simulink model "pvwindupfc11"  (R2016a)
settings: Solver=VariableStepAuto  StartTime=0.0  StopTime=0.5  RelTol=1e-3
undefined symbols (not defined in the file): BCMS11, c1, c2, c3, c4, c5, c6, Clink_3L, DiscIntNeverNeededParam, fdesignblkfcn, Fnom, gcbh, Ion, Ki_Ireg_3L, Ki_VDCreg_3L, Kp_Ireg_3L, Kp_VDCreg_3L, LimitL_Ireg_3L, LimitL_VDCreg_3L, LimitU_Ireg_3L, LimitU_VDCreg_3L, Lithium, LowerLimit, Pnom_3L, Pnom_dc_3L, PV11, Ts_Control, Ts_Power, Ts_PWM, UpperLimit, Vnom_dc_3L, Vnom_prim_3L, Vnom_sec_3L
libraries: powerlib x98, powerlib_extras x29, powerlib_meascontrol x20, fuzblock x2, simulink x1, electricdrivelib x1
(part 2 of 4)

== system pvwindupfc11/100Vdc DC//DC Converter1 ==
  Add : Sum
  CBus : powerlib/Elements/Series RLC Branch  LConnTagsString=__new0  RConnTagsString=__new0  BranchType=RC  Resistance=0.2  Inductance=1e-3  SetiL0=off  InitialCurrent=0  Capacitance=7500e-6  Setx0=on  InitialVoltage=100  Measurements=None
  Chopper : Subsystem  mask(SPSdrives Converter){SnubberResistance=10e3, SnubberCapacitance=inf, Ron=1e-3, ForwardVoltages=[1.3,1.3], IGBTParameters=[0,0], converterType=Inverter}
      mask prompts: SnubberResistance "Snubber resistance Rs (Ohms):"; SnubberCapacitance "Snubber capacitance Cs (F):"; Ron "Ron (Ohms):"; ForwardVoltages "Forward voltages [Device Vf(V), Diode Vd (V)]"; IGBTParameters "[Tf(s), Tt(s)]:"; converterType "Converter type:"
      mask help: This model implements an average-value buck converter."Duty Cycle" contains the duty cycle of the internal IGBT device.
      mask TypeOptions converterType: Rectifier | Inverter
      mask Display: plot(0,0,100,100,[39 39 23.8],[71 28 28],[44 56 49.6 56 52.8 56 61 61],[39.2 33.6 32.8 33.6 40.8 33.6 30 12.4],[44 44 44 61 61],[28 71 60 66.4 90],[75 67 83 75 67 83 75 75],[54 42 42 54 54 54 54 66],[61 75 75],[24 24 42],[75 75 61],[66,76,76])
  Constant : Constant  Value=100
  Current controller DISCRETE1 : Subsystem  mask(PI controller){Kp=0.0005, Ki=0.15, Ts=1e-3}
      mask prompts: Kp "Proportional gain (Kp)"; Ki "Integral gain (Ki)"; Ts "Sample time (s) :"
      mask help: Proportional-Integral Speed Controller
      mask Display: plot(0,0,100,100,[35,35,65],[70,30,30],[35,65],[45,60])
  Current controller DISCRETE2 : Subsystem  mask(PI controller){Kp=0.0005, Ki=0.15, Ts=1e-3}
      mask prompts: Kp "Proportional gain (Kp)"; Ki "Integral gain (Ki)"; Ts "Sample time (s) :"
      mask help: Proportional-Integral Speed Controller
      mask Display: plot(0,0,100,100,[35,35,65],[70,30,30],[35,65],[45,60])
  Duty Cycles : Subsystem
  L : powerlib/Elements/Series RLC Branch  LConnTagsString=__new0  RConnTagsString=__new0  BranchType=L  Resistance=0.3  Inductance=500e-6  SetiL0=off  InitialCurrent=0  Capacitance=100e-6  Setx0=off  InitialVoltage=0  Measurements=None
  Timer : Subsystem  DialogController=POWERSYS.PowerSysDialog  mask(Timer){t=[ 0  1], e=[1 1 ]}
      mask prompts: t "Time (s):"; e "Amplitude:"
      mask help:
      | Generates a signal changing at specified times.
      |
      | If a signal value is not specified at time zero, the output is kept at 0 until the first specified transition time.
      mask init:
      | tt=t;
      | sv=e;
      | if isempty(tt) | isempty(sv)
      | 	% probably during the load process when under a masked block.
      | 	tt=0;
      | 	sv=1;
      | end
      | %
      | if length(sv) ~= length(tt),
      |    Erreur.message = 'The vectors specifying the time and amplitude pairs must have the same length.';
      |    Erreur.identifier = 'SimPowerSystems:TimerBlock:ParameterError';
      |    powericon('psberror',Erreur.message,Erreur.identifier,'NoUiwait');
      | end
      | if tt(1)~=0,
      |    tt=[0 tt];
      |    sv=[~sv(1) sv];
      | end
      | n=length(tt);
      | vec_dt=[tt,0]-[0,tt] ;
      | vec_dt=vec_dt(2:n);
      | if any(vec_dt<=0)
      |    Erreur.message = 'All transition times must be in increasing order.';
      |    Erreur.identifier = 'SimPowerSystems:TimerBlock:ParameterError';
      |    powericon('psberror',Erreur.message,Erreur.identifier,'NoUiwait');
      | end
      | tv=[-1,tt(1),reshape(repmat(reshape(tt(2:end),1,length(tt)-1),2,1),1,2*length(tt)-2),tt(end)+1];
      | %sv=(sv(:)'~=0);
      | opv=[sv(1),reshape(repmat(sv(1:end-1),2,1),1,2*length(sv)-2),sv(end),sv(end)];
      | 
      | power_initmask();
      mask Help: web(psbhelp)
      mask Display: plot( tv(2:end-1), opv(2:end-1) )
  Transfer Fcn : TransferFcn  Denominator=[0.001 1]
  Voltage Measurement : powerlib/Measurements/Voltage Measurement  PhasorSimulation=off  OutputType=Complex  PSBequivalent=0
  + : PMIOPort  Tag=PMCPort  Port=1  Side=Right
  - : PMIOPort  Tag=PMCPort  Port=2  Side=Right
  + input : PMIOPort  Tag=PMCPort  Port=3  Side=Left
  -input : PMIOPort  Tag=PMCPort  Port=4  Side=Left
  wires:
  Transfer Fcn/1 -> Current controller DISCRETE1/1(UBus)
  Duty Cycles/1(dc) -> Chopper/1(Duty Cycle)
  Voltage Measurement/1 -> Transfer Fcn/1
  Constant/1 -> Current controller DISCRETE1/2(Uref)
  Timer/1(Out) -> Current controller DISCRETE2/1(Pref)
  [Ppv] -> Current controller DISCRETE2/2(Ppv)
  Current controller DISCRETE2/1(Delta Ec) -> Add/2
  Add/1 -> Duty Cycles/1(Ec)
  Current controller DISCRETE1/1(Ec) -> Add/1
  connections:
  + input/RConn1 -- L/RConn1
  Chopper/RConn1 -- L/LConn1
  CBus/LConn1 -- Chopper/LConn1 -- +/RConn1 -- Voltage Measurement/LConn1
  Chopper/LConn2 -- CBus/RConn1 -- -/RConn1 -- Voltage Measurement/LConn2 -- -input/RConn1

== system pvwindupfc11/60 kW  PV Array 1 ==
  note: Diode characteristic
      |    Id=Isat*[exp(Vd/VT) -1]
      |
      | where:
      |    Id = diode cuurent (A)
      |    Vd = diode voltage (V)
      |  Isat = diode saturation current (A)
      |    VT = temperature voltage = k*T/q*Qd*Ncell*Nser
      |
      |     T = cell temperature (K),
      |     k = Boltzman constant = 1.3806e-23 J.K^-1
      |     q = electron charge = 1.6022e-19 C
      |    Qd = diode quality factor
      |  Ncell= number of series-connected cells per module
      |  Nser = number of series-connected modules per string
  Ir : Inport
  Add : Sum  Inputs=+-
  Bus Creator : BusCreator  Inputs=4
  Diode : Subsystem
      mask Display:
      | plot(-75,-50,100,150, [-15 -15 43 -15 -15 -75],[50 8 50 92 50 50], ...
      |     [43 43],[8 94],[100 43], [50 50])
  I_PV : powerlib/Measurements/Current Measurement  PhasorSimulation=off  OutputType=Complex  PSBequivalent=0
  Iph : powerlib/Electrical Sources/Controlled Current Source  Initialize=on  Source_Type=AC  Amplitude=0  Phase=0  Frequency=0  Measurements=None
  Iph_ : Constant  Value=Iph_array
  Product1 : Product  Inputs=**  RndMeth=Zero
  Rp : powerlib/Elements/Series RLC Branch  LConnTagsString=__new0  RConnTagsString=__new0  BranchType=R  Resistance=Rp_array  Inductance=1e-3  SetiL0=off  InitialCurrent=0  Capacitance=1e-6  Setx0=off  InitialVoltage=0  Measurements=Branch current
  Rs : powerlib/Elements/Series RLC Branch  LConnTagsString=__new0  RConnTagsString=__new0  BranchType=R  Resistance=Rs_array  Inductance=1e-3  SetiL0=off  InitialCurrent=0  Capacitance=1e-6  Setx0=off  InitialVoltage=0  Measurements=None
  Rs_ : Gain  Gain=Rs_array
  t0_kW : Gain  Gain=1e-3
  + : PMIOPort  Port=1  Side=Right
  - : PMIOPort  Port=2  Side=Right
  m : Outport
  wires:
  Product1/1 -> Iph/1
  Iph_/1 -> Product1/1
  Ir/1 -> t0_kW/1, Bus Creator/4  "Irradiance (W/m^2)"
  Diode/1(Vdiode) -> Add/1  "Vdiode"
  Rs_/1 -> Add/2
  I_PV/1 -> Rs_/1, Bus Creator/2  "I_PV"
  t0_kW/1 -> Product1/2
  Add/1 -> Bus Creator/1  "V_PV"
  Diode/2(Idiode) -> Bus Creator/3  "I_diode"
  Bus Creator/1 -> m/1
  connections:
  Iph/LConn1 -- Diode/RConn1 -- -/RConn1 -- Rp/RConn1
  Diode/LConn1 -- Iph/RConn1 -- Rs/RConn1 -- Rp/LConn1
  Rs/LConn1 -- I_PV/LConn1
  +/RConn1 -- I_PV/RConn1

== system pvwindupfc11/Control Systems  ==
  REC Control : Subsystem
  SEC Control : Subsystem

== system pvwindupfc11/Control of Inverter ==
  note: Control of Inverter
  Discrete PWM Generator1 : Subsystem  AncestorBlock=|  DialogController=POWERSYS.PowerSysDialog  mask(Discrete PWM Generator){GeneratorMode=3-arm  bridge (6 pulses), Fc=4000, Ts=50e-6, Internal=off, mIndex=0.99, Freq=50, Phase=0}
      | powerlib_extras/Discrete 
      | Control Blocks/Discrete
      | PWM Generator
      mask prompts: GeneratorMode "Generator Mode"; Fc "Carrier frequency (Hz):"; Ts "Sample time:"; Internal "Internal generation of modulating signal(s)"; mIndex "Modulation index  (0<m<1) :"; Freq "Frequency of output voltage (Hz)"; Phase "Phase of output voltage (degrees)"
      mask help:
      | This discrete block generates pulses for carrier-based PWM (Pulse Width Modulation), self-commutated IGBTs,GTOs or FETs bridges.
      |
      | Depending on the number of bridge arms selected in the "Generator Mode" parameter, the block can be used either for single-phase or three-phase PWM control.
      mask init:
      | powericon('psbcallbacks',gcb,'Discrete PWM Generator');
      | if Freq==0
      |     Phase=90;
      | end
      | switch GeneratorMode
      | case 1,
      |     Internal_Phase=0;
      |    Signal_PortWidth=1;
      |    Select1_Elements=[1 2];
      |    Select1_PortWidth=2;
      |    Select3_Elements=[1 2];
      |    Select3_PortWidth=4;
      | case 2,
      |     Internal_Phase=0;
      |     Signal_PortWidth=1;
      |     Select1_Elements=[1 2];
      |     Select1_PortWidth=2;
      |     Select3_Elements=[1 2 3 4];
      |     Select3_PortWidth=4;
      | case 3,
      |     Internal_Phase=[0 -2*pi/3 2*pi/3];
      |     Signal_PortWidth=3;
      |     Select1_Elements=[1 4 2 5 3 6];
      |     Select1_PortWidth=6;
      |    Select3_Elements=[1 2 3 4 5 6];
      |    Select3_PortWidth=12;
      | case 4,
      |     Internal_Phase=[0 -2*pi/3 2*pi/3];
      |     Signal_PortWidth=3;
      |     Select1_Elements=[1 4 2 5 3 6];
      |     Select1_PortWidth=6;
      |    Select3_Elements=[1 2 3 4 5 6 7 8 9 10 11 12];
      |    Select3_PortWidth=12;
      | end
      | power_initmask();
      mask Help:
      | The output pulses are a vector (with values=0 or 1). Depending on the selected "Generator Mode", the output vector contains:
      | For a 1-arm  bridge: Two pulses. Pulse 1 is for the upper switch and pulse 2 is for the lower switch.
      | For a 2-arm  bridge: Four pulses. Pulses 1 and 3 are respectively for the upper switches of the first and second arm. Pulses 2 and 4 are for the lower switches.
      | For a 3-arm  bridge: Six pulses. Pulses 1,3 and 5 are respectively for the upper switches of the first,second and third arm. Pulses 2,4 and 6 are for the lower switches.
      | For double 3-arm bridges: Twelve pulses.The first six pulses (pulses 1 to 6) must be sent to the first 3-arm bridge and the last six (pulses 7 to 12) to the second 3-arm bridge.
      | 
      | By selecting "Internal generation" you can can control the modulation index m, frequency and phase of the output voltage  from the internal parameters (m, Freq and Phase). Otherwise, external signals are used for pulse generation. The width of the input vector must be 1 for single phase bridges ( 1-arm or 2-arm)  and 3 for 3-phase bridges  (single or double bridge).
      mask TypeOptions GeneratorMode: 1-arm  bridge (2 pulses) | 2-arm  bridge (4 pulses) | 3-arm  bridge (6 pulses) | Double 3-arm  bridges (12 pulses)
      mask Callback Internal: powericon('psbcallbacks',gcb,'Discrete PWM Generator',[]);
  MI Controller : Subsystem
  Subsystem1 : Subsystem
  Unit Delay4 : UnitDelay  SampleTime=20e-6
  VL-L : Scope
  Vph_rms : Scope
  m : Scope
  C : PMIOPort  Port=1  Side=Left
  B : PMIOPort  Port=2  Side=Left
  A : PMIOPort  Port=3  Side=Left
  Pulses : Outport
  wires:
  MI Controller/2(m) -> m/1
  Unit Delay4/1 -> Pulses/1
  Subsystem1/1(Vph) -> MI Controller/1(Vabc)
  Subsystem1/2(VL-L) -> VL-L/1
  Subsystem1/3(Vph_rms) -> Vph_rms/1
  Discrete PWM Generator1/1(Pulses) -> Unit Delay4/1
  MI Controller/1(Vabc_inv) -> Discrete PWM Generator1/1(Uref)
  connections:
  A/RConn1 -- Subsystem1/LConn1
  B/RConn1 -- Subsystem1/LConn2
  C/RConn1 -- Subsystem1/LConn3

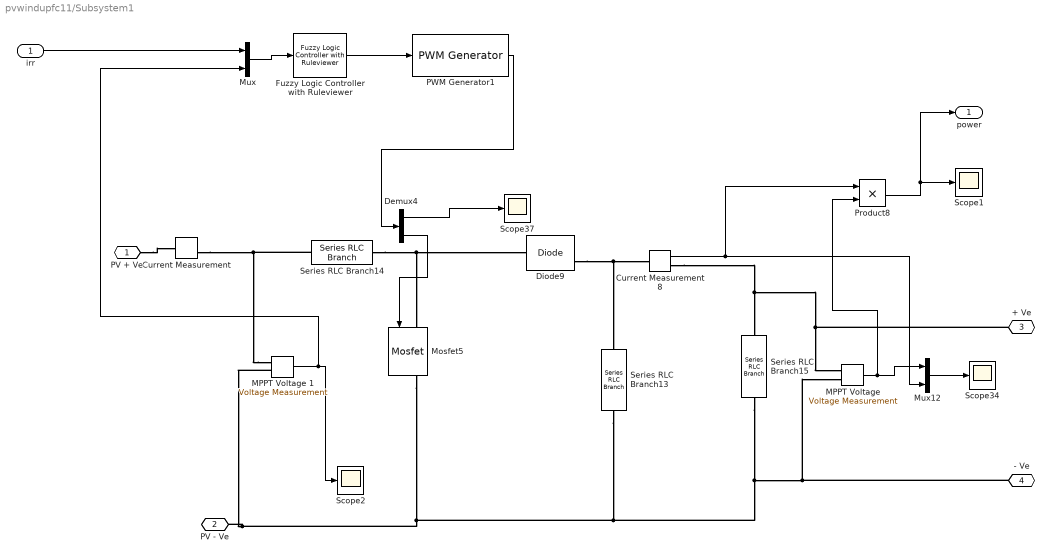
== system pvwindupfc11/Subsystem1 ==
  irr : Inport
  Current Measurement : powerlib/Measurements/Current Measurement  PhasorSimulation=off  OutputType=Complex  PSBequivalent=0
  Current Measurement8 : powerlib/Measurements/Current Measurement  PhasorSimulation=off  OutputType=Complex  PSBequivalent=0
  Demux4 : Demux  Outputs=2
  Diode9 : powerlib/Power Electronics/Diode  Ron=0.001  Lon=0  Vf=0.8  IC=0  UseSnubber=off  Rs=500  Cs=250e-9  Measurements=on
  Fuzzy Logic Controller with Ruleviewer : fuzblock/Fuzzy Logic  Controller  with Ruleviewer  fismatrix=[PV11]  Ts=0.01
  "MPPT Voltage " : powerlib/Measurements/Voltage Measurement  PhasorSimulation=off  OutputType=Complex  PSBequivalent=0
  MPPT Voltage 1 : powerlib/Measurements/Voltage Measurement  PhasorSimulation=off  OutputType=Complex  PSBequivalent=0
  Mosfet5 : powerlib/Power Electronics/Mosfet  Ron=0.1  Lon=0  Rd=0.01  Vfd=0  IC=0  Rs=1e5  Cs=inf  Measurements=on
  Mux : Mux  Inputs=2
  Mux12 : Mux  Inputs=2
  PWM Generator1 : powerlib_extras/Control  Blocks/PWM Generator  GeneratorMode="1-arm  bridge (2 pulses)"  Fc=2000  Internal=off  mIndex=0.4  Freq=50  Phase=0
  Product8 : Product  RndMeth=Zero
  Scope{1..2,34,37} (4 alike) : Scope
  Series RLC Branch13 : powerlib/Elements/Series RLC Branch  LConnTagsString=__new0  RConnTagsString=__new0  BranchType=C  Resistance=1  Inductance=1e-3  SetiL0=off  InitialCurrent=0  Capacitance=15.5e-4  Setx0=off  InitialVoltage=0  Measurements=None
  Series RLC Branch14 : powerlib/Elements/Series RLC Branch  LConnTagsString=__new0  RConnTagsString=__new0  BranchType=L  Resistance=1  Inductance=0.05e-2  SetiL0=off  InitialCurrent=0  Capacitance=1e-6  Setx0=off  InitialVoltage=0  Measurements=None
  Series RLC Branch15 : powerlib/Elements/Series RLC Branch  LConnTagsString=__new0  RConnTagsString=__new0  BranchType=R  Resistance=55  Inductance=1e-3  SetiL0=off  InitialCurrent=0  Capacitance=1e-6  Setx0=off  InitialVoltage=0  Measurements=None
  PV + Ve : PMIOPort  Port=1  Side=Left
  PV - Ve : PMIOPort  Port=2  Side=Left
  + Ve : PMIOPort  Port=3  Side=Right
  - Ve : PMIOPort  Port=4  Side=Right
  "power " : Outport
  wires:
  Demux4/2 -> Mosfet5/1
  PWM Generator1/1 -> Demux4/1
  Demux4/1 -> Scope37/1
  Mux12/1 -> Scope34/1
  "MPPT Voltage "/1 -> Product8/2, Mux12/1
  Current Measurement8/1 -> Product8/1, Mux12/2
  Product8/1 -> "power "/1, Scope1/1
  MPPT Voltage 1/1 -> Mux/2, Scope2/1
  Fuzzy Logic Controller with Ruleviewer/1 -> PWM Generator1/1
  Mux/1 -> Fuzzy Logic Controller with Ruleviewer/1
  irr/1 -> Mux/1
  connections:
  MPPT Voltage 1/LConn1 -- Series RLC Branch14/LConn1 -- Current Measurement/RConn1
  MPPT Voltage 1/LConn2 -- PV - Ve/RConn1 -- Series RLC Branch13/RConn1 -- - Ve/RConn1 -- "MPPT Voltage "/LConn2 -- Series RLC Branch15/RConn1 -- Mosfet5/RConn1
  + Ve/RConn1 -- Series RLC Branch15/LConn1 -- Current Measurement8/RConn1 -- "MPPT Voltage "/LConn1
  Diode9/RConn1 -- Current Measurement8/LConn1 -- Series RLC Branch13/LConn1
  Series RLC Branch14/RConn1 -- Diode9/LConn1 -- Mosfet5/LConn1
  PV + Ve/RConn1 -- Current Measurement/LConn1

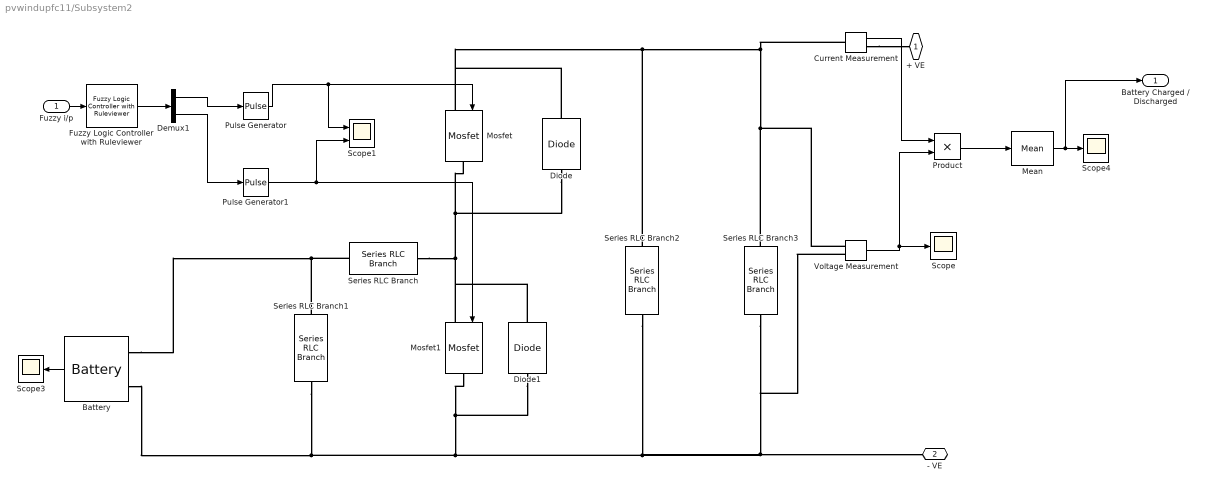
== system pvwindupfc11/Subsystem2 ==
  Fuzzy i/p : Inport
  Battery : electricdrivelib/Extra Sources/Battery  BatType=Lithium-Ion  ShowTempParam=off  ThermalPreset=no  NomV=440  NomQ=30  SOC=100  Batt_Tr=1  PresetModel=off  MaxQ=30  MinV=330  FullV=512.1543  Dis_rate=13.0435  R=0.14667  Normal_OP=27.1304  expZone="[475.3698      1.473913]"  current=[6.5 13 32.5]  Units=Time  Tci=20  NomT=25  T2=0  MaxQ2=2.208  FullV2=3.45  Normal_OP2=2.8  expZone2="[3.22        0.23]"  Rca=0.6  ti=1000  Dp=0
  Current Measurement : powerlib/Measurements/Current Measurement  PhasorSimulation=off  OutputType=Complex  PSBequivalent=0
  Demux1 : Demux  Outputs=2
  Diode : powerlib/Power Electronics/Diode  Ron=0.001  Lon=0  Vf=0.8  IC=0  UseSnubber=off  Rs=500  Cs=250e-9  Measurements=off
  Diode1 : powerlib/Power Electronics/Diode  Ron=0.001  Lon=0  Vf=0.8  IC=0  UseSnubber=off  Rs=500  Cs=250e-9  Measurements=off
  Fuzzy Logic Controller with Ruleviewer : fuzblock/Fuzzy Logic  Controller  with Ruleviewer  fismatrix=[BCMS11]  Ts=0.1
  Mean : powerlib_meascontrol/Measurements/Mean  Freq=60  Vinit=0  Ts=0
  Mosfet : powerlib/Power Electronics/Mosfet  Ron=0.1  Lon=0  Rd=0.01  Vfd=0  IC=0  Rs=1e5  Cs=inf  Measurements=off
  Mosfet1 : powerlib/Power Electronics/Mosfet  Ron=0.1  Lon=0  Rd=0.01  Vfd=0  IC=0  Rs=1e5  Cs=inf  Measurements=off
  Product : Product
  Pulse Generator : DiscretePulseGenerator  PulseType=Time based  TimeSource=Use external signal  Period=0.01  PulseWidth=99  PhaseDelay=0.001
  Pulse Generator1 : DiscretePulseGenerator  PulseType=Time based  TimeSource=Use external signal  Period=0.01  PulseWidth=99  PhaseDelay=0.001
  Scope : Scope
  Scope1 : Scope  NumInputPorts=2
  Scope3 : Scope
  Scope4 : Scope
  Series RLC Branch : powerlib/Elements/Series RLC Branch  LConnTagsString=__new0  RConnTagsString=__new0  BranchType=L  Resistance=1  Inductance=100e-6  SetiL0=off  InitialCurrent=0  Capacitance=1e-6  Setx0=off  InitialVoltage=0  Measurements=None
  Series RLC Branch1 : powerlib/Elements/Series RLC Branch  LConnTagsString=__new0  RConnTagsString=__new0  BranchType=RC  Resistance=1  Inductance=1e-3  SetiL0=off  InitialCurrent=0  Capacitance=700e-4  Setx0=off  InitialVoltage=0  Measurements=None
  Series RLC Branch2 : powerlib/Elements/Series RLC Branch  LConnTagsString=__new0  RConnTagsString=__new0  BranchType=RC  Resistance=2  Inductance=1e-3  SetiL0=off  InitialCurrent=0  Capacitance=700e-4  Setx0=off  InitialVoltage=0  Measurements=None
  Series RLC Branch3 : powerlib/Elements/Series RLC Branch  LConnTagsString=__new0  RConnTagsString=__new0  BranchType=R  Resistance=0.3  Inductance=1e-3  SetiL0=off  InitialCurrent=0  Capacitance=1e-6  Setx0=off  InitialVoltage=0  Measurements=None
  Voltage Measurement : powerlib/Measurements/Voltage Measurement  PhasorSimulation=off  OutputType=Complex  PSBequivalent=0
  + VE : PMIOPort  Port=1  Side=Right
  - VE : PMIOPort  Port=2  Side=Right
  "Battery Charged / Discharged " : Outport
  wires:
  Battery/1 -> Scope3/1
  Fuzzy Logic Controller with Ruleviewer/1 -> Demux1/1
  Demux1/1 -> Pulse Generator/1
  Demux1/2 -> Pulse Generator1/1
  Voltage Measurement/1 -> Product/2, Scope/1
  Pulse Generator1/1 -> Scope1/2, Mosfet1/1
  Pulse Generator/1 -> Scope1/1, Mosfet/1
  Fuzzy i/p/1 -> Fuzzy Logic Controller with Ruleviewer/1
  Current Measurement/1 -> Product/1
  Product/1 -> Mean/1
  Mean/1 -> "Battery Charged / Discharged "/1, Scope4/1
  connections:
  Series RLC Branch/RConn1 -- Mosfet1/LConn1 -- Diode1/RConn1 -- Diode/LConn1 -- Mosfet/RConn1
  Series RLC Branch/LConn1 -- Series RLC Branch1/LConn1 -- Battery/LConn1
  Mosfet1/RConn1 -- Diode1/LConn1 -- Battery/LConn2 -- Series RLC Branch1/RConn1 -- Series RLC Branch2/RConn1 -- Series RLC Branch3/RConn1 -- Voltage Measurement/LConn2 -- - VE/RConn1
  Series RLC Branch3/LConn1 -- Current Measurement/LConn1 -- Diode/RConn1 -- Mosfet/LConn1 -- Series RLC Branch2/LConn1 -- Voltage Measurement/LConn1
  Current Measurement/RConn1 -- + VE/RConn1

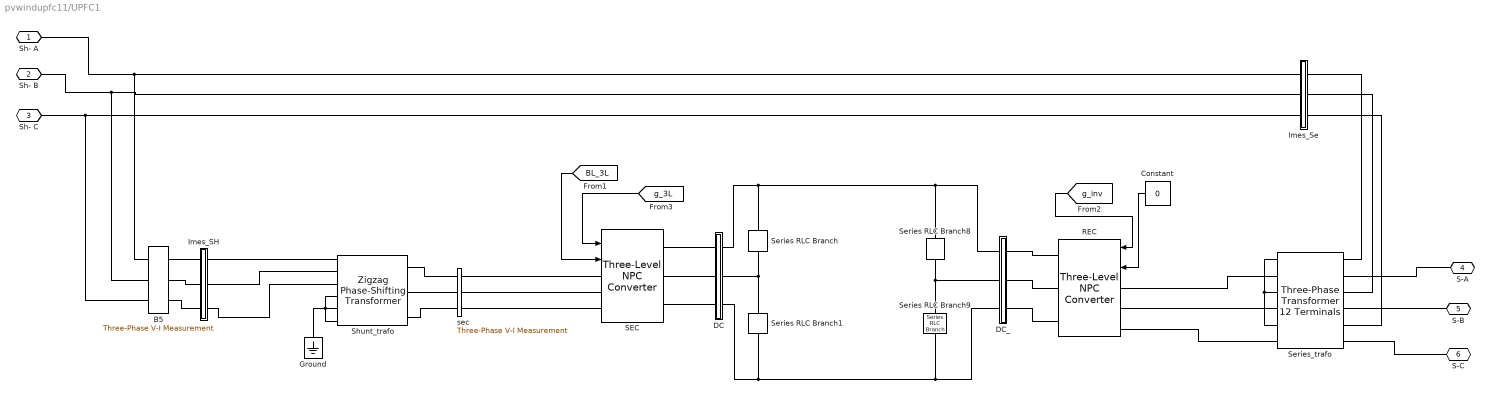
== system pvwindupfc11/UPFC1 ==
  B5 : powerlib/Measurements/Three-Phase V-I Measurement  VoltageMeasurement=phase-to-phase  SetLabelV=on  LabelV=V_shunt  Vpu=off  VpuLL=off  CurrentMeasurement=yes  SetLabelI=on  LabelI=i_shunt_  Ipu=off  Pbase=100e6  Vbase=500e3  OutputType=Complex  PhasorSimulation=off  PSBequivalent=0
  Constant : Constant  Value=0
  DC : Subsystem
  DC_ : Subsystem
  Ground : powerlib/Elements/Ground  LConnTagsString=a
  Imes_SH : Subsystem
  Imes_Se : Subsystem
  REC : powerlib/Power Electronics/Three-Level NPC Converter  ModelType=Switching devices  Ron=1e-3  Rs=1e6  Cs=inf  Vforward=[0,0]  Ron_Diode=1e-3  Rs_Diode=1e6  Cs_Diode=inf  Vf_Diode=1e-3  Rs_CurrentSource=inf
  SEC : powerlib/Power Electronics/Three-Level NPC Converter  ModelType=Switching devices  Ron=1e-3  Rs=1e6  Cs=inf  Vforward=[ 0, 0 ]  Ron_Diode=1e-3  Rs_Diode=1e6  Cs_Diode=inf  Vf_Diode=1e-3  Rs_CurrentSource=inf
      settings: AttributesFormatString=%<ModelType>
  Series RLC Branch : powerlib/Elements/Series RLC Branch  LConnTagsString=__new0  RConnTagsString=__new0  BranchType=C  Resistance=1  Inductance=1e-3  SetiL0=off  InitialCurrent=0  Capacitance=Clink_3L  Setx0=on  InitialVoltage=Vc_Initial_3L  Measurements=None
  Series RLC Branch1 : powerlib/Elements/Series RLC Branch  LConnTagsString=__new0  RConnTagsString=__new0  BranchType=C  Resistance=1  Inductance=1e-3  SetiL0=off  InitialCurrent=0  Capacitance=Clink_3L  Setx0=on  InitialVoltage=Vc_Initial_3L  Measurements=None
  Series RLC Branch8 : powerlib/Elements/Series RLC Branch  LConnTagsString=__new0  RConnTagsString=__new0  BranchType=C  Resistance=1  Inductance=1e-3  SetiL0=off  InitialCurrent=0  Capacitance=Clink_3L  Setx0=on  InitialVoltage=Vc_Initial_3L  Measurements=None
  Series RLC Branch9 : powerlib/Elements/Series RLC Branch  LConnTagsString=__new0  RConnTagsString=__new0  BranchType=C  Resistance=1  Inductance=1e-3  SetiL0=off  InitialCurrent=0  Capacitance=Clink_3L  Setx0=off  InitialVoltage=1000  Measurements=None
  Series_trafo : powerlib/Elements/Three-Phase Transformer 12 Terminals  RatedPower="[Pnom_3L,  Fnom ]"  Winding1="[Vnom_sec_3L   0.002  0.1/2]"  Winding2="[Vnom_sec_3L   0.002  0.1/2]"  RmXm=[ 500 500 ]
  Shunt_trafo : powerlib/Elements/Zigzag Phase-Shifting Transformer  SecondaryConnection=Y  UNITS=SI  NominalPower="[Pnom_3L,  Fnom ]"  PrimaryVoltage=Vnom_prim_3L  SecondaryVoltage="[Vnom_sec_3L   1]"  Winding1=[1.0624 0.084547]  Winding2=[0.00042304 3.3664e-05]  Winding3=[0.0004 3.1831e-05]  SetSaturation=off  RmLm=[3.1873e+05 3.1873e+05]  Rm=3.1873e+05  Saturation=[0 0;0.077613 65.62;32.339 83.118]  SetInitialFlux=off  Measurements=None  InitialFluxes=[0 0 0]  MoreParameters=off  BreakLoop=off  DataType=on
      settings: AttributesFormatString=\n
  sec : powerlib/Measurements/Three-Phase V-I Measurement  VoltageMeasurement=phase-to-phase  SetLabelV=on  LabelV=Vsec_3L_LL  Vpu=off  VpuLL=off  CurrentMeasurement=no  SetLabelI=on  LabelI=Isec  Ipu=off  Pbase=100e6  Vbase=500e3  OutputType=Complex  PhasorSimulation=off  PSBequivalent=0
  Sh- A : PMIOPort  Port=1  Side=Left
  Sh- B : PMIOPort  Port=2  Side=Left
  Sh- C : PMIOPort  Port=3  Side=Left
  S-A : PMIOPort  Port=4  Side=Right
  S-B : PMIOPort  Port=5  Side=Right
  S-C : PMIOPort  Port=6  Side=Right
  wires:
  [g_3L] -> SEC/1
  [BL_3L] -> SEC/2
  Constant/1 -> REC/2
  [g_inv] -> REC/1
  connections:
  Sh- B/RConn1 -- B5/LConn2 -- Imes_Se/LConn2
  Series RLC Branch9/RConn1 -- DC_/LConn3 -- DC/RConn3 -- Series RLC Branch1/RConn1
  Sh- C/RConn1 -- B5/LConn3 -- Imes_Se/LConn3
  S-B/RConn1 -- Series_trafo/RConn4
  Imes_SH/RConn3 -- Shunt_trafo/LConn3
  S-C/RConn1 -- Series_trafo/RConn6
  sec/RConn3 -- Shunt_trafo/RConn3
  Imes_SH/RConn2 -- Shunt_trafo/LConn2
  Series RLC Branch/RConn1 -- DC/RConn2 -- Series RLC Branch1/LConn1
  Series RLC Branch/LConn1 -- Series RLC Branch8/LConn1 -- DC_/LConn1 -- DC/RConn1
  B5/RConn1 -- Imes_SH/LConn1
  Series_trafo/LConn6 -- REC/LConn3
  sec/RConn2 -- Shunt_trafo/RConn2
  sec/RConn1 -- Shunt_trafo/RConn1
  Series_trafo/LConn2 -- REC/LConn1
  Sh- A/RConn1 -- B5/LConn1 -- Imes_Se/LConn1
  DC_/RConn3 -- REC/RConn3
  Imes_Se/RConn2 -- Series_trafo/RConn3
  Series_trafo/LConn3 -- Series_trafo/LConn5 -- Series_trafo/LConn1
  sec/LConn2 -- SEC/LConn2
  sec/LConn1 -- SEC/LConn1
  Imes_Se/RConn1 -- Series_trafo/RConn1
  B5/RConn3 -- Imes_SH/LConn3
  DC_/RConn2 -- REC/RConn2
  Imes_Se/RConn3 -- Series_trafo/RConn5
  SEC/RConn3 -- DC/LConn3
  sec/LConn3 -- SEC/LConn3
  S-A/RConn1 -- Series_trafo/RConn2
  SEC/RConn1 -- DC/LConn1
  Imes_SH/RConn1 -- Shunt_trafo/LConn1
  SEC/RConn2 -- DC/LConn2
  DC_/RConn1 -- REC/RConn1
  Series RLC Branch8/RConn1 -- Series RLC Branch9/LConn1 -- DC_/LConn2
  Series_trafo/LConn4 -- REC/LConn2
  Shunt_trafo/LConn5 -- Shunt_trafo/LConn6 -- Ground/LConn1 -- Shunt_trafo/LConn4
  B5/RConn2 -- Imes_SH/LConn2

== system pvwindupfc11/Wind-MPPT ==
  wm : Inport
  Ia : Inport  Port=2
  Vd : Inport  Port=3
  Current Controller1 : Subsystem  mask{h=0.1}
      mask prompts: h "Hysteresis band (A)"
      mask help: Hysteresis Current Controller
      mask Display: plot(0,0,100,100,[45,45],[35,65],[55,55],[35,65],[45,65],[65,65],[35,55],[35,35])
  Discrete 1st-Order Filter2 : powerlib_extras/Discrete  Control Blocks/Discrete 1st-Order Filter  FilterType=Lowpass  Tc=100e-3  Ts=20e-6  Initialize=off  Vac_Init=[0.8 -25 60]  Vdc_Init=-0.4  PlotResponse=off  param1=[1 500 0.1]
  Subsystem : Subsystem
  Torque reference 1 : Subsystem
  Unit Delay3 : UnitDelay  SampleTime=-1
  genertaor terminal1 : Scope  NumInputPorts=2
  p : Outport
  wires:
  Unit Delay3/1 -> Current Controller1/2(Ia)
  Torque reference 1/1(Tref) -> Subsystem/1(Tref)
  Subsystem/1(Id_ref) -> Discrete 1st-Order Filter2/1
  Discrete 1st-Order Filter2/1 -> Current Controller1/1(Iref)
  Current Controller1/1(g) -> p/1, genertaor terminal1/1
  wm/1 -> Torque reference 1/1(wm), Subsystem/2(wm)
  Vd/1 -> Subsystem/3(Vd)
  Ia/1 -> Unit Delay3/1
  Current Controller1/2(error1) -> genertaor terminal1/2

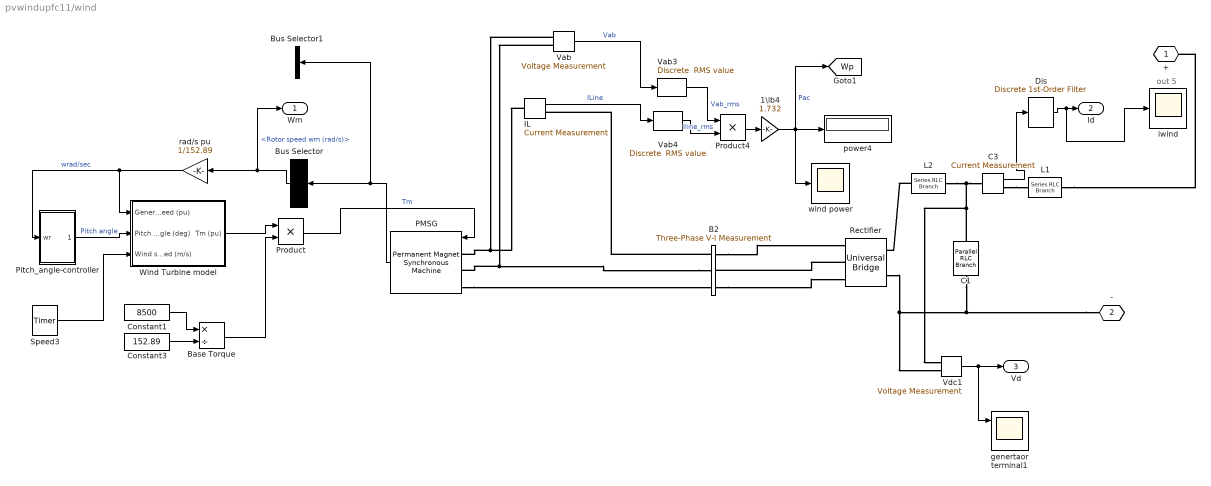
== system pvwindupfc11/wind ==
  note: out 5
  1\ib4 : Gain  Gain=1.732  SaturateOnIntegerOverflow=on  OutDataTypeStr=Inherit: Same as input  ParamDataTypeStr=Inherit: Same as input
  "B2 " : powerlib/Measurements/Three-Phase V-I Measurement  VoltageMeasurement=no  SetLabelV=on  LabelV=Vabc_B2  Vpu=off  VpuLL=off  CurrentMeasurement=no  SetLabelI=on  LabelI=Iabc_B2  Ipu=off  Pbase=100e6  Vbase=500e3  OutputType=Magnitude  PhasorSimulation=off  PSBequivalent=0
  Base Torque : Product  Inputs=*/  RndMeth=Zero
  Bus Selector : BusSelector  OutputSignals=Rotor speed wm (rad/s)
  Bus Selector1 : BusSelector  OutputSignals=Rotor speed wm (rad/s)
  C1 : powerlib/Elements/Parallel RLC Branch  LConnTagsString=a  RConnTagsString=__new0  BranchType=C  Resistance=1.0  Inductance=1.0  SetiL0=off  InitialCurrent=0  Capacitance=1000e-06  Setx0=off  InitialVoltage=650  Measurements=None
  C3 : powerlib/Measurements/Current Measurement  PhasorSimulation=off  OutputType=Complex  PSBequivalent=0
  Constant1 : Constant  Value=8500
  Constant3 : Constant  Value=152.89
  Dis : powerlib_extras/Discrete  Control Blocks/Discrete 1st-Order Filter  FilterType=Lowpass  Tc=100e-3  Ts=20e-6  Initialize=off  Vac_Init=[0.8 -25 60]  Vdc_Init=-0.4  PlotResponse=off  param1=[1 500 0.1]
  IL : powerlib/Measurements/Current Measurement  PhasorSimulation=off  OutputType=Complex  PSBequivalent=0
  L1 : powerlib/Elements/Series RLC Branch  LConnTagsString=__new0  RConnTagsString=__new0  BranchType=L  Resistance=1.0  Inductance=2e-3  SetiL0=off  InitialCurrent=0  Capacitance=1.0  Setx0=off  InitialVoltage=0  Measurements=None
  L2 : powerlib/Elements/Series RLC Branch  LConnTagsString=__new0  RConnTagsString=__new0  BranchType=L  Resistance=1.0  Inductance=2e-3  SetiL0=off  InitialCurrent=0  Capacitance=1.0  Setx0=off  InitialVoltage=0  Measurements=None
  PMSG : powerlib/Machines/Permanent Magnet Synchronous Machine  NbPhases=3  FluxDistribution=Sinusoidal  RotorType=Round  MechanicalLoad=Torque Tm  PresetModel=No  ShowDetailedParameters=on  MeasurementBus=off  Resistance=0.425  Inductance=8.5e-3  dqInductances=[0.0082 0.0082]  La=0.000395  MachineConstant=Flux linkage established by magnets (V.s)  Flux=0.433  VoltageCst=392.6876  TorqueCst=3.2475  Flat=120  Mechanical=[0.01197 0.001189 5]  PolePairs=5  InitialConditions=[0,0, 0,0]  InitialConditions5ph=[0 0 0 0 0 0]  TsPowergui=0  TsBlock=-1  RefAngle=90 degrees behind phase A axis (modified Park)
  Pitch_angle-controller : Subsystem
  Product : Product  RndMeth=Zero
  Product4 : Product  RndMeth=Zero
  Rectifier : powerlib/Power Electronics/Universal Bridge  Arms=3  SnubberResistance=100  SnubberCapacitance=0.1e-6  Device=Diodes  Ron=1e-3  Lon=0  ForwardVoltages="[  0.8  0.8  ]"  ForwardVoltage=.8  GTOparameters=[ 10e-6 , 20e-6 ]  IGBTparameters=[ 1e-6 , 2e-6 ]  Measurements=Device currents  Measurements_2=None  converterType=Rectifier
  Speed3 : powerlib_extras/Control  Blocks/Timer  t=[0 .5 3]  e=[5 12 9]
  Vab : powerlib/Measurements/Voltage Measurement  PhasorSimulation=off  OutputType=Complex  PSBequivalent=0
  Vab3 : powerlib_extras/Discrete Measurements/Discrete  RMS value  Freq=50  Mag_Init=0  Ts=20e-6
  Vab4 : powerlib_extras/Discrete Measurements/Discrete  RMS value  Freq=50  Mag_Init=0  Ts=20e-6
  Vdc1 : powerlib/Measurements/Voltage Measurement  Tag=PoWeRsYsTeMmEaSuReMeNt  PhasorSimulation=off  OutputType=Magnitude  PSBequivalent=0
  Wind Turbine model : Subsystem  AncestorBlock=DRlib/Wind Generation/Wind Turbine  DialogController=POWERSYS.PowerSysDialog  mask(Wind Turbine){Pnom=8.5e3, Pelec_base=8.5e3/0.9, wind_base=12, P_wind_base=0.8, speed_nom=1, pitch_angle=0, DisplayTurbChar=off, c1_c6=[0.51763          116          0.4            5           21     0.006795], cp_nom=0.48, lambda_nom=8.1}
      mask prompts: Pnom "Nominal mechanical output power (W):"; Pelec_base "Base power of the electrical generator (VA):"; wind_base "Base wind speed (m/s):"; P_wind_base "Maximum power at base wind speed (pu of nominal mechanical power):"; speed_nom "Base rotational speed (p.u. of base generator speed):"; pitch_angle "Pitch angle beta to display wind-turbine power characteristics (beta >=0)  (deg):"; DisplayTurbChar "Display wind turbine power characteristics"
      mask help:
      | This block implements a variable pitch wind turbine model. The performance coefficient Cp of the turbine is the mechanical output power of the turbine divided by wind power and a function of wind speed, rotational speed, and pitch angle (beta). Cp reaches its maximum value at zero beta. Select the wind-turbine power characteristics display to plot the turbine characteristics at the specified pitch angle.
      |
      | The first input is the generator speed in per unit of the generator base speed. For a synchronous or asynchronous generator, the base speed is the synchronous speed. For a permanent-magnet generator, the base speed is defined as the speed producing nominal voltage at  no load. The second input is the blade pitch angle (beta) in degrees. The third input is the wind speed in m/s.
      |
      | The output is the torque applied to the generator shaft in per unit of the generator ratings.
      |
      | The turbine inertia must be added to the generator inertia.
      mask init:
      | %Wind turbine typical characteristic data
      | %c2=116;c3=0.4;c4=5;c5=21;
      | %Computation of c1 and c6 for lambda_nom et cpmax
      | %lambda_nom=8.1;
      | %cp_max=0.48;
      | %cp_nom=cp_max;
      | 
      | %lambda_i_nom=1/(1/lambda_nom-0.035);
      | %k_nom=-(c2*c5/lambda_i_nom-c4*c5-c2)*exp(-c5/lambda_i_nom)/lambda_nom^2;
      | %c1=cp_max/((c2/lambda_i_nom-c4)*exp(-c5/lambda_i_nom)+k_nom*lambda_nom);
      | %c6=k_nom*c1;
      | power_initmask();
      mask Help: web(psbhelp);
      mask Callback Pnom:
      | ParVisible={'on','on','on','on','on','on','on','off','off','off',};
      | set_param(gcb,'MaskVisibilities',ParVisible);
      | c1_c6=str2num(get_param(gcb,'c1_c6'));
      | c1=c1_c6(1);c2=c1_c6(2);c3=c1_c6(3);c4=c1_c6(4);c5=c1_c6(5);c6=c1_c6(6);
      mask Callback DisplayTurbChar:
      | DisplayTurbChar=get_param(gcb,'DisplayTurbChar');
      | 
      | if strcmp(DisplayTurbChar,'on')
      |     fig_num=figure;
      | 	clf(fig_num);
      | 	[speed_nom,wind_base,P_wind_base,pitch_angle]=getSPSmaskvalues(gcb,{'speed_nom','wind_base','P_wind_base','pitch_angle'});
      | 	[c1_c6,lambda_nom,cp_nom]=getSPSmaskvalues(gcb,{'c1_c6','lambda_nom','cp_nom'});
      | 	c1=c1_c6(1);c2=c1_c6(2);c3=c1_c6(3);c4=c1_c6(4);c5=c1_c6(5);c6=c1_c6(6);
      | 
      | 	%Wind turbine typical characteristic data
      |     %c2=116;c3=0.4;c4=5;c5=21;
      |     %Computation of c1 and c6 for lambda_nom et cpmax
      |     %lambda_nom=8.1;
      |     %cp_max=0.48;
      |     %cp_nom=cp_max;
      | 
      |     %lambda_i_nom=1/(1/lambda_nom-0.035);
      |     %k_nom=-(c2*c5/lambda_i_nom-c4*c5-c2)*exp(-c5/lambda_i_nom)/lambda_nom^2;
      |     %c1=cp_max/((c2/lambda_i_nom-c4)*exp(-c5/lambda_i_nom)+k_nom*lambda_nom);
      |     %c6=k_nom*c1;
      | 
      | 	wr_elec_pu=1e-3:0.01:1.5;;
      |     wr_mec_pu=wr_elec_pu/speed_nom;
      |     wind_max=ceil((1.2/P_wind_base)^(1/3)*wind_base);
      |     wind_min=round(((0.1)/P_wind_base)^(1/3)*wind_base);
      |     wind1=wind_min:(wind_base-wind_min)/5:wind_base;
      |     wind2=wind_base+(wind_base-wind_min)/5:(wind_base-wind_min)/5:wind_max;
      |     wind_pu=[wind1 wind2]/wind_base;
      | 
      |     for k=1:length(wind_pu)
      |         for i=1:length(wr_mec_pu);
      |             lambda_pu=wr_mec_pu(i)/wind_pu(k);
      |             lambda=lambda_pu*lambda_nom;
      |             lambda_i=1/(1/(lambda+0.08*pitch_angle)-0.035/(pitch_angle^3+1));
      |             cp=c1*(c2/lambda_i-c3*pitch_angle-c4)*exp(-c5/lambda_i)+c6*lambda;
      |             cp_pu=cp/cp_nom;
      |             Pwind_pu(k,i)=wind_pu(k)^3*cp_pu*P_wind_base;
      |         end
      |     end
      |     for k=1:length(wind_pu)
      |         plot(wr_elec_pu,Pwind_pu(k,:))
      |         hold on
      |     end
      | 
      |     plot([speed_nom,speed_nom,0],[0,P_wind_base,P_wind_base],'r--')
      |     text(speed_nom+0.01,0+0.05,sprintf('%0.4g pu',speed_nom))
      |     text(0.01,P_wind_base+0.05,sprintf('Max. power at base wind speed (%0.4g m/s) and beta = 0 deg',wind_base))
      |     for i=1:length(wind_pu),
      |         p_max(i)=max(Pwind_pu(i,:));
      |         speed(i)=wr_elec_pu(find(Pwind_pu(i,:)==p_max(i)));
      |         text(speed(i),p_max(i),sprintf('%0.4g m/s',wind_pu(i)*wind_base))
      |     end
      |     plot([0 max(wr_elec_pu)],[0 0],'--')
      | 
      |     xlabel('Turbine speed (pu of nominal generator speed)')
      |     ylabel('Turbine output power (pu of nominal mechanical power)')
      |     title(sprintf('Turbine Power Characteristics (Pitch angle beta = %0.4g deg)',pitch_angle))
      |     axis([0 max(wr_elec_pu) min(Pwind_pu(1,:)) max(P_wind_base+0.1,max(wind_pu)^3*P_wind_base+0.1)])
      |     set_param(gcb,'DisplayTurbChar','off')
      | end
      mask Display: disp('');
  genertaor terminal1 : Scope  NumInputPorts=2
  iwind : Scope
  power4 : Display
      settings: SampleTime=1e-3
  rad/s pu : Gain  Gain=1/152.89  SaturateOnIntegerOverflow=on  OutDataTypeStr=Inherit: Same as input  ParamDataTypeStr=Inherit: Same as input
  wind power : Scope
  + : PMIOPort  Tag=PMCPort  Port=1  Side=Right
  - : PMIOPort  Tag=PMCPort  Port=2  Side=Right
  Wm : Outport
  Id : Outport  Port=2
  Vd : Outport  Port=3
  tag scope: Wp=global
  wires:
  Wind Turbine model/1(Tm (pu)) -> Product/1
  Constant1/1 -> Base Torque/1
  Constant3/1 -> Base Torque/2
  Bus Selector/1 -> rad/s pu/1, Wm/1  "<Rotor speed wm (rad/s)>"
  rad/s pu/1 -> Wind Turbine model/1(Generator speed (pu)), Pitch_angle-controller/1(wr)  "wrad/sec"
  Vab/1 -> Vab3/1  "Vab"
  IL/1 -> Vab4/1  "ILine"
  Product4/1 -> 1\ib4/1
  Product/1 -> PMSG/1  "Tm"
  Vab3/1 -> Product4/1  "Vab_rms"
  Vab4/1 -> Product4/2  "Iline_rms"
  1\ib4/1 -> power4/1, wind power/1, [Wp]  "Pac"
  Base Torque/1 -> Product/2
  Vdc1/1 -> genertaor terminal1/1, Vd/1
  Pitch_angle-controller/1(Pitch_angle) -> Wind Turbine model/2(Pitch angle (deg))  "Pitch angle"
  Speed3/1 -> Wind Turbine model/3(Wind speed (m/s))
  PMSG/1 -> Bus Selector/1, Bus Selector1/1
  C3/1 -> Dis/1
  Dis/1 -> Id/1, iwind/1
  connections:
  "B2 "/LConn1 -- IL/RConn1
  "B2 "/LConn2 -- PMSG/LConn2 -- Vab/LConn2
  PMSG/LConn3 -- "B2 "/LConn3
  "B2 "/RConn1 -- Rectifier/LConn1
  Rectifier/LConn2 -- "B2 "/RConn2
  "B2 "/RConn3 -- Rectifier/LConn3
  -/RConn1 -- C1/RConn1 -- Vdc1/LConn2 -- Rectifier/RConn2
  C3/LConn1 -- Vdc1/LConn1 -- C1/LConn1 -- L2/RConn1
  C3/RConn1 -- L1/LConn1
  Vab/LConn1 -- IL/LConn1 -- PMSG/LConn1
  L2/LConn1 -- Rectifier/RConn1
  L1/RConn1 -- +/RConn1

== system pvwindupfc11/100Vdc DC//DC Converter1/Chopper ==
  Duty Cycle : Inport
  Average-value armature voltage : Fcn  Expr=u(1)*u(2)
  Average-value source current : Fcn  Expr=u(1)*u(2)
  Controlled Current Source : powerlib/Electrical Sources/Controlled Current Source  Initialize=on  Source_Type=AC  Amplitude=0  Phase=0  Frequency=0  Measurements=None
  Controlled Voltage Source : powerlib/Electrical Sources/Controlled Voltage Source  Initialize=on  Source_Type=AC  Amplitude=0  Phase=0  Frequency=0  Measurements=None
  Current Measurement : powerlib/Measurements/Current Measurement  Tag=PoWeRsYsTeMmEaSuReMeNt  PhasorSimulation=off  OutputType=Magnitude  PSBequivalent=0
  Memory : Memory
  Memory1 : Memory
  Mux : Mux  Inputs=2
  Mux1 : Mux  Inputs=2
  Selector : Selector  InputPortWidth=2  IndexOptions=Index vector (dialog)  Indices=[1]  OutputSizes=1
  Voltage Measurement1 : powerlib/Measurements/Voltage Measurement  Tag=PoWeRsYsTeMmEaSuReMeNt  PhasorSimulation=off  OutputType=Magnitude  PSBequivalent=0
  A : PMIOPort  Port=1  Side=Right
  + : PMIOPort  Port=2  Side=Left
  - : PMIOPort  Port=3  Side=Left
  wires:
  Memory/1 -> Controlled Voltage Source/1
  Average-value armature voltage/1 -> Memory/1
  Mux/1 -> Average-value armature voltage/1
  Voltage Measurement1/1 -> Mux/2
  Duty Cycle/1 -> Selector/1
  Mux1/1 -> Average-value source current/1
  Current Measurement/1 -> Mux1/2
  Average-value source current/1 -> Memory1/1
  Memory1/1 -> Controlled Current Source/1
  Selector/1 -> Mux/1, Mux1/1
  connections:
  Voltage Measurement1/LConn2 -- Controlled Current Source/RConn1 -- -/RConn1 -- Controlled Voltage Source/LConn1
  Controlled Current Source/LConn1 -- Voltage Measurement1/LConn1 -- +/RConn1
  Controlled Voltage Source/RConn1 -- Current Measurement/LConn1
  A/RConn1 -- Current Measurement/RConn1

== system pvwindupfc11/100Vdc DC//DC Converter1/Current controller DISCRETE1 ==
  UBus : Inport
  Uref : Inport  Port=2
  Ctrl sat. : Saturate  UpperLimit=0.95  LowerLimit=-0.95
  Discrete-Time Integrator : DiscreteIntegrator  IntegratorMethod=Integration: Trapezoidal  SampleTime=Ts  LimitOutput=on  UpperSaturationLimit=0.95  LowerSaturationLimit=-0.95  ICPrevOutput=DiscIntNeverNeededParam  ICPrevScaledInput=DiscIntNeverNeededParam
  Integral gain : Gain  Gain=Ki  SaturateOnIntegerOverflow=on  OutDataTypeStr=Inherit: Same as input  ParamDataTypeStr=Inherit: Same as input
  Proportional gain : Gain  Gain=Kp  SaturateOnIntegerOverflow=on  OutDataTypeStr=Inherit: Same as input  ParamDataTypeStr=Inherit: Same as input
  Sum1 : Sum  Inputs=+-  SaturateOnIntegerOverflow=on  InputSameDT=on  OutDataTypeStr=Inherit: Same as first input
  Sum2 : Sum  SaturateOnIntegerOverflow=on  InputSameDT=on  OutDataTypeStr=Inherit: Same as first input
  Ec : Outport  InitialOutput=0
  wires:
  Proportional gain/1 -> Sum2/1
  Integral gain/1 -> Discrete-Time Integrator/1
  Sum1/1 -> Integral gain/1, Proportional gain/1
  UBus/1 -> Sum1/1
  Uref/1 -> Sum1/2
  Discrete-Time Integrator/1 -> Sum2/2
  Sum2/1 -> Ctrl sat./1
  Ctrl sat./1 -> Ec/1

== system pvwindupfc11/100Vdc DC//DC Converter1/Current controller DISCRETE2 ==
  Pref : Inport
  Ppv : Inport  Port=2
  Ctrl sat. : Saturate  UpperLimit=0.95  LowerLimit=-0.95
  Discrete-Time Integrator : DiscreteIntegrator  IntegratorMethod=Integration: Trapezoidal  SampleTime=Ts  LimitOutput=on  UpperSaturationLimit=0.95  LowerSaturationLimit=-0.95  ICPrevOutput=DiscIntNeverNeededParam  ICPrevScaledInput=DiscIntNeverNeededParam
  Integral gain : Gain  Gain=Ki  SaturateOnIntegerOverflow=on  OutDataTypeStr=Inherit: Same as input  ParamDataTypeStr=Inherit: Same as input
  Proportional gain : Gain  Gain=Kp  SaturateOnIntegerOverflow=on  OutDataTypeStr=Inherit: Same as input  ParamDataTypeStr=Inherit: Same as input
  Sum1 : Sum  Inputs=+-  SaturateOnIntegerOverflow=on  InputSameDT=on  OutDataTypeStr=Inherit: Same as first input
  Sum2 : Sum  SaturateOnIntegerOverflow=on  InputSameDT=on  OutDataTypeStr=Inherit: Same as first input
  Delta Ec : Outport  InitialOutput=0
  wires:
  Ctrl sat./1 -> Delta Ec/1
  Sum2/1 -> Ctrl sat./1
  Discrete-Time Integrator/1 -> Sum2/2
  Ppv/1 -> Sum1/2
  Pref/1 -> Sum1/1
  Sum1/1 -> Proportional gain/1, Integral gain/1
  Integral gain/1 -> Discrete-Time Integrator/1
  Proportional gain/1 -> Sum2/1

== system pvwindupfc11/100Vdc DC//DC Converter1/Duty Cycles ==
  Ec : Inport
  Add : Sum  Inputs=+-
  Bus Creator2 : BusCreator  Inputs=2
  Constant : Constant
  Duty Cycle : Fcn  Expr=0.5*(u[1]+1)
  dc : Outport
  wires:
  Duty Cycle/1 -> Add/2, Bus Creator2/1  "IGBT I"
  Add/1 -> Bus Creator2/2  "IGBT 2"
  Constant/1 -> Add/1
  Ec/1 -> Duty Cycle/1
  Bus Creator2/1 -> dc/1

== system pvwindupfc11/100Vdc DC//DC Converter1/Timer ==
  Clock : Clock
  Derivative : Derivative
  Hit Crossing : HitCross  ShowOutputPort=off
  Look-Up Table : Lookup  InputValues=tv  Table=opv  SaturateOnIntegerOverflow=on
  Out : Outport
  wires:
  Clock/1 -> Look-Up Table/1
  Look-Up Table/1 -> Out/1, Derivative/1
  Derivative/1 -> Hit Crossing/1

== system pvwindupfc11/60 kW  PV Array 1/Diode ==
  note: Id=Isat*[exp(Vd/Vt)-1]
  Add : Sum  Inputs=+-
  Id : powerlib/Electrical Sources/Controlled Current Source  Initialize=on  Source_Type=AC  Amplitude=0  Phase=0  Frequency=0  Measurements=None
  Is : Constant  Value=Isat_array
  Math Function : Math  SaturateOnIntegerOverflow=on
  Product : Product  RndMeth=Zero
  Product1 : Product  Inputs=*/  RndMeth=Zero
  VT : Constant  Value=VT_array
  Vd : powerlib/Measurements/Voltage Measurement  PhasorSimulation=off  OutputType=Complex  PSBequivalent=0
  one : Constant
  A : PMIOPort  Port=1  Side=Left
  K : PMIOPort  Port=2  Side=Right
  Vdiode : Outport
  Idiode : Outport  Port=2
  wires:
  VT/1 -> Product1/2
  Add/1 -> Product/2
  one/1 -> Add/2
  Product1/1 -> Math Function/1
  Is/1 -> Product/1  "Is"
  Vd/1 -> Vdiode/1, Product1/1
  Product/1 -> Id/1, Idiode/1
  Math Function/1 -> Add/1
  connections:
  Id/LConn1 -- A/RConn1 -- Vd/LConn1
  Vd/LConn2 -- K/RConn1 -- Id/RConn1

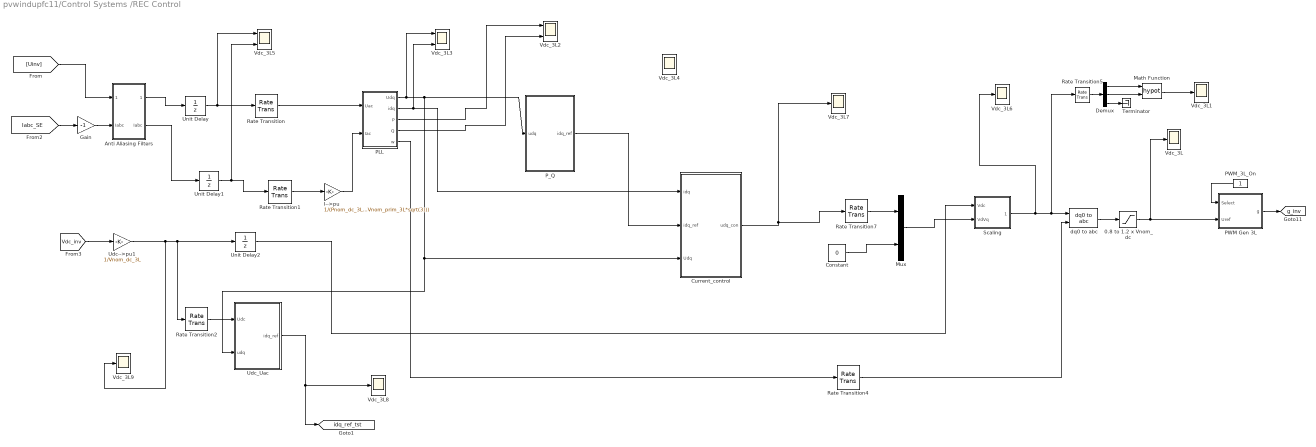
== system pvwindupfc11/Control Systems /REC Control ==
  0.8 to 1.2 x Vnom_dc : Saturate  UpperLimit=1.5  LowerLimit=0
  Anti Aliasing Filters : Subsystem  mask(Anti-aliasing (2nd order lowpass)){Fc=800, Ts=1e-6}
      mask prompts: Fc "Cut-off frequency (Hz):"; Ts "Sample time:"
  Constant : Constant  Value=0  SampleTime=1e-6
  Current_control : Subsystem
  Demux : Demux  Outputs=3
  Gain : Gain  Gain=-1
  I-->pu : Gain  Gain=1/(Pnom_dc_3L*sqrt(2)/(Vnom_prim_3L*sqrt(3)))
  Math Function : Math  Operator=hypot  SaturateOnIntegerOverflow=on
  Mux : Mux  Inputs=2
  PLL : Subsystem
  PWM Gen 3L : Subsystem
  PWM_3L_On : Constant
      settings: AttributesFormatString=%<Tag>
  P_Q : Subsystem
  Rate Transition{,1..2,5} (4 alike) : RateTransition  OutPortSampleTime=Ts_Control
  Rate Transition4 : RateTransition  OutPortSampleTime=Ts_PWM
  Rate Transition7 : RateTransition  OutPortSampleTime=Ts_PWM
  Scaling : Subsystem
  Terminator : Terminator
  Udc-->pu1 : Gain  Gain=1/Vnom_dc_3L
  Udc_Uac : Subsystem
  Unit Delay : UnitDelay  SampleTime=Ts_Power
  Unit Delay1 : UnitDelay  SampleTime=Ts_Power
  Unit Delay2 : UnitDelay  SampleTime=Ts_PWM
  Vdc_3L{,1,4,6..9} (7 alike) : Scope
  Vdc_3L2 : Scope  NumInputPorts=2
  Vdc_3L3 : Scope  NumInputPorts=2
  Vdc_3L5 : Scope  NumInputPorts=2
  dq0 to abc : powerlib_meascontrol/Transformations/dq0 to abc  Alignment=90 degrees behind phase A axis
  tag scope: g_inv=global, idq_ref_tst=global
  wires:
  [Vdc_inv] -> Udc-->pu1/1
  Anti Aliasing Filters/2(Iabc) -> Unit Delay1/1
  Rate Transition1/1 -> I-->pu/1
  Unit Delay/1 -> Vdc_3L5/1, Rate Transition/1
  Rate Transition/1 -> PLL/1(Uac)
  Unit Delay1/1 -> Vdc_3L5/2, Rate Transition1/1
  I-->pu/1 -> PLL/2(Iac)
  PLL/4(Q) -> Vdc_3L2/2
  PLL/2(idq) -> Vdc_3L3/2, Current_control/1(idq)
  PLL/1(Udq) -> Vdc_3L3/1, Current_control/3(Udq), Udc_Uac/2(udq), P_Q/1(udq)
  Current_control/1(udq_con) -> Vdc_3L7/1, Rate Transition7/1
  Constant/1 -> Mux/2
  PWM Gen 3L/1(g) -> [g_inv]
  PWM_3L_On/1 -> PWM Gen 3L/1(Select)
  dq0 to abc/1 -> 0.8 to 1.2 x Vnom_dc/1
  Scaling/1(VdVq*) -> Vdc_3L6/1, Rate Transition5/1, dq0 to abc/1
  Demux/3 -> Terminator/1
  Demux/2 -> Math Function/2
  Demux/1 -> Math Function/1
  Rate Transition5/1 -> Demux/1
  Math Function/1 -> Vdc_3L1/1
  PLL/5(w) -> Rate Transition4/1
  Mux/1 -> Scaling/2(VdVq)
  Rate Transition4/1 -> dq0 to abc/2
  Unit Delay2/1 -> Scaling/1(Vdc)
  Rate Transition7/1 -> Mux/1
  [Uinv] -> Anti Aliasing Filters/1(Vabc)
  Anti Aliasing Filters/1(" Vabc") -> Unit Delay/1
  [Iabc_SE] -> Gain/1
  Gain/1 -> Anti Aliasing Filters/2("Iabc ")
  Udc-->pu1/1 -> Vdc_3L9/1, Unit Delay2/1, Rate Transition2/1
  Rate Transition2/1 -> Udc_Uac/1(Udc)
  Udc_Uac/1(idq_ref) -> [idq_ref_tst], Vdc_3L8/1
  0.8 to 1.2 x Vnom_dc/1 -> Vdc_3L/1, PWM Gen 3L/2(Uref)
  PLL/3(P) -> Vdc_3L2/1
  P_Q/1(idq_ref) -> Current_control/2(idq_ref)

== system pvwindupfc11/Control Systems /SEC Control ==
  Block1 : Step  Time=999  SampleTime=Ts_Power
  I->pu2 : Gain  SaturateOnIntegerOverflow=on  OutDataTypeStr=Inherit: Same as input  ParamDataTypeStr=Inherit: Same as input
  PWM Gen 3L : Subsystem
  PWM_3L_On : Constant
      settings: AttributesFormatString=%<Tag>
  SEC Control System : Subsystem
  Unit Delay : UnitDelay  SampleTime=Ts_Power
  Unit Delay1 : UnitDelay  SampleTime=Ts_Power
  Unit Delay2 : UnitDelay  SampleTime=Ts_Power
  tag scope: BL_3L=global, Uref_3L=global, g_3L=global, meas_3L=global
  wires:
  SEC Control System/2(meas) -> [meas_3L]
  Block1/1 -> [BL_3L]
  [Vgrid] -> Unit Delay/1
  SEC Control System/1(Uref abc) -> [Uref_3L], PWM Gen 3L/2(Uref)
  [Vdc_3L] -> Unit Delay2/1
  Unit Delay1/1 -> SEC Control System/2(Igrid)
  Unit Delay2/1 -> SEC Control System/3(Vdc)
  Unit Delay/1 -> SEC Control System/1(Vgrid)
  PWM Gen 3L/1(g) -> [g_3L]
  PWM_3L_On/1 -> PWM Gen 3L/1(Select)
  I->pu2/1 -> Unit Delay1/1
  [Iabc_SH] -> I->pu2/1

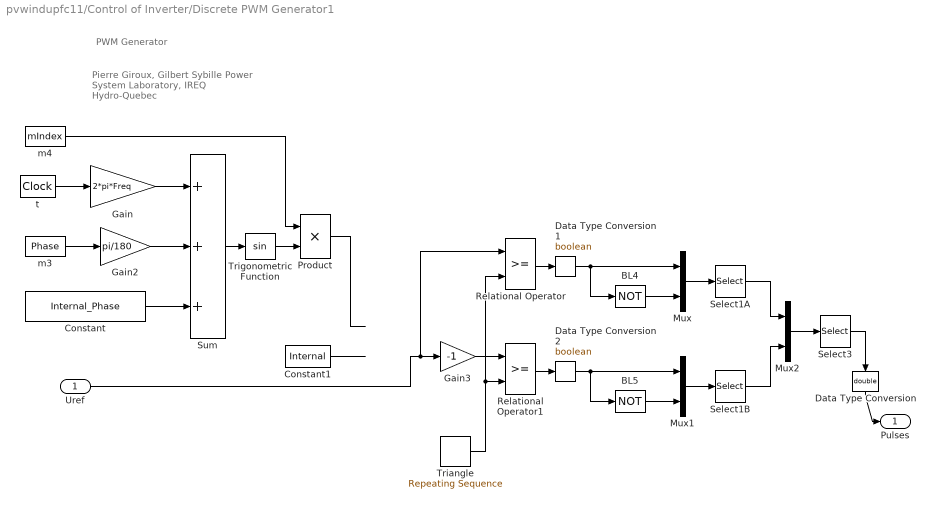
== system pvwindupfc11/Control of Inverter/Discrete PWM Generator1 ==
  note: Pierre Giroux, Gilbert Sybille
      | Power System Laboratory, IREQ
      | Hydro-Quebec
  note: PWM Generator
  Uref : Inport
  BL4 : Logic  Operator=NOT  Inputs=1
  BL5 : Logic  Operator=NOT  Inputs=1
  Constant : Constant  Value=Internal_Phase
  Constant1 : Constant  Value=Internal
  Data Type Conversion : DataTypeConversion  OutDataTypeStr=double  SaturateOnIntegerOverflow=on  RndMeth=Zero
  Data Type Conversion1 : DataTypeConversion  OutDataTypeStr=boolean  SaturateOnIntegerOverflow=on  RndMeth=Zero
  Data Type Conversion2 : DataTypeConversion  OutDataTypeStr=boolean  SaturateOnIntegerOverflow=on  RndMeth=Zero
  Gain : Gain  Gain=2*pi*Freq  SaturateOnIntegerOverflow=on  OutDataTypeStr=Inherit: Same as input  ParamDataTypeStr=Inherit: Same as input
  Gain2 : Gain  Gain=pi/180  SaturateOnIntegerOverflow=on  OutDataTypeStr=Inherit: Same as input  ParamDataTypeStr=Inherit: Same as input
  Gain3 : Gain  Gain=-1  SaturateOnIntegerOverflow=on  OutDataTypeStr=Inherit: Same as input  ParamDataTypeStr=Inherit: Same as input
  Mux : Mux  Inputs=2
  Mux1 : Mux  Inputs=2
  Mux2 : Mux  Inputs=2
  Product : Product  SaturateOnIntegerOverflow=on  InputSameDT=on  OutDataTypeStr=Inherit: Same as first input
  Relational Operator : RelationalOperator  InputSameDT=on
  Relational Operator1 : RelationalOperator  InputSameDT=on
  Select1A : Selector  InputPortWidth=Select1_PortWidth  IndexOptions=Index vector (dialog)  Indices=Select1_Elements  OutputSizes=1
  Select1B : Selector  InputPortWidth=Select1_PortWidth  IndexOptions=Index vector (dialog)  Indices=Select1_Elements  OutputSizes=1
  Select3 : Selector  InputPortWidth=Select3_PortWidth  IndexOptions=Index vector (dialog)  Indices=Select3_Elements  OutputSizes=1
  Sum : Sum  Inputs=+++  SaturateOnIntegerOverflow=on  InputSameDT=on  OutDataTypeStr=Inherit: Same as first input
  Triangle : simulink/Sources/Repeating Sequence  rep_seq_t=[0 1/Fc/4 3/Fc/4 1/Fc]  rep_seq_y=[0 -1 1 0]
  Trigonometric Function : Trigonometry
  m3 : Constant  Value=Phase
  m4 : Constant  Value=mIndex
  t : DigitalClock  SampleTime=Ts
  Pulses : Outport
  wires:
  Mux2/1 -> Select3/1
  Select1B/1 -> Mux2/2
  Select1A/1 -> Mux2/1
  Mux1/1 -> Select1B/1
  Mux/1 -> Select1A/1
  BL5/1 -> Mux1/2
  BL4/1 -> Mux/2
  Gain3/1 -> Relational Operator1/1
  Triangle/1 -> Relational Operator1/2, Relational Operator/2
  Product/1 -> ?
  Constant1/1 -> ?
  Uref/1 -> Relational Operator/1, Gain3/1
  Trigonometric Function/1 -> Product/2
  Sum/1 -> Trigonometric Function/1
  m4/1 -> Product/1
  Constant/1 -> Sum/3
  m3/1 -> Gain2/1
  Gain2/1 -> Sum/2
  Gain/1 -> Sum/1
  t/1 -> Gain/1
  Select3/1 -> Data Type Conversion/1
  Data Type Conversion/1 -> Pulses/1
  Relational Operator/1 -> Data Type Conversion1/1
  Data Type Conversion1/1 -> BL4/1, Mux/1
  Relational Operator1/1 -> Data Type Conversion2/1
  Data Type Conversion2/1 -> BL5/1, Mux1/1
